simulink model "estimator"  (R2025b)
settings: configuration reference "cfgEstimator" (kept outside this file)
undefined symbols (not defined in the file or in its folder): BMS_iRest, BMS_ocvSoc, BMS_ocvV, BMS_Qnom, BMS_socMismatchTol, BMS_tRelax, BMS_tRestRecal, BMS_Ts
libraries: simulink x4
settings Model: DataDictionary=estimator.sldd  Creator=SC-Br  LastModifiedBy=SC-Br
settings ConfigSetRef: SourceName=cfgEstimator

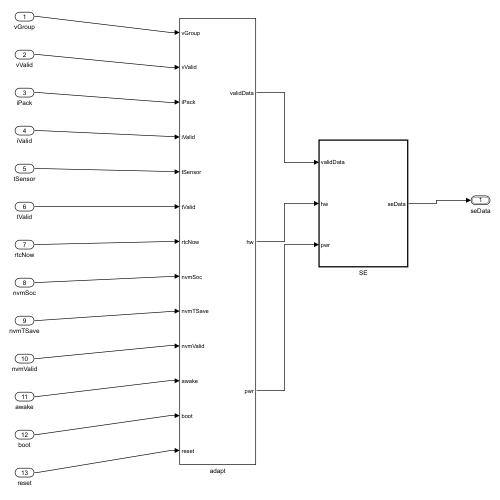
[thumbnail: Simulink's stored preview of the top-level diagram]
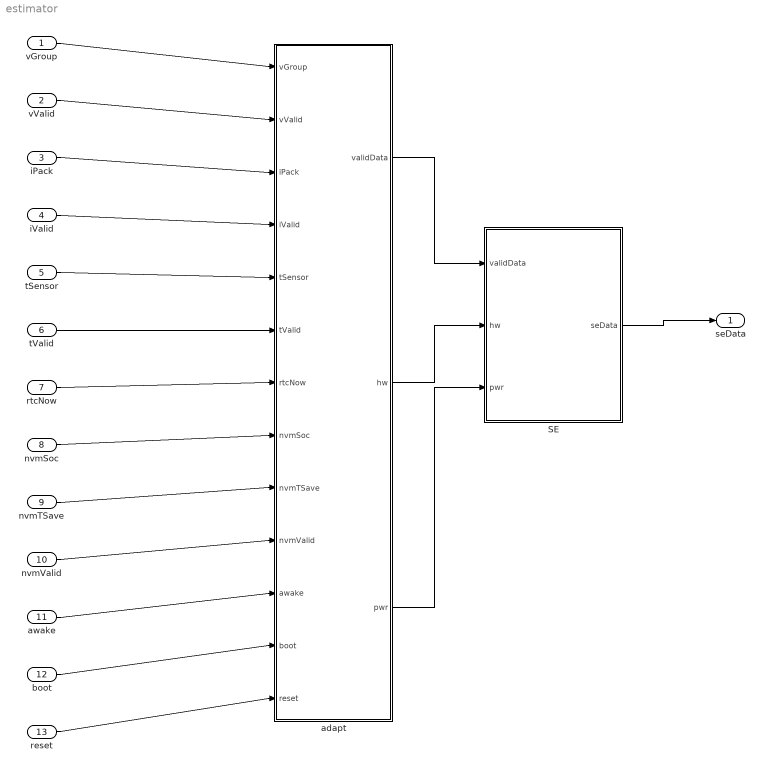
== system estimator ==
  vGroup : Inport  Description=Group voltages from f_CellVoltages (V)  OutDataTypeStr=double  PortDimensions=13  SampleTime=BMS_Ts
  vValid : Inport  Description=Not f_CellVoltages invalid flag  Port=2  OutDataTypeStr=boolean  PortDimensions=13  SampleTime=BMS_Ts
  iPack : Inport  Description=Pack current from f_PackValuesP0 (A, discharge positive)  Port=3  OutDataTypeStr=double  PortDimensions=1  SampleTime=BMS_Ts
  iValid : Inport  Description=Current received and plausible  Port=4  OutDataTypeStr=boolean  PortDimensions=1  SampleTime=BMS_Ts
  tSensor : Inport  Description=Temperatures from f_CellTemperatures (K)  Port=5  OutDataTypeStr=double  PortDimensions=26  SampleTime=BMS_Ts
  tValid : Inport  Description=Not f_CellTemperatures invalid flag  Port=6  OutDataTypeStr=boolean  PortDimensions=26  SampleTime=BMS_Ts
  rtcNow : Inport  Description=Pi clock (s, same epoch as nvmTSave)  Port=7  OutDataTypeStr=double  PortDimensions=1  SampleTime=BMS_Ts
  nvmSoc : Inport  Description=SOC record file: group SOC  Port=8  OutDataTypeStr=double  PortDimensions=13  SampleTime=BMS_Ts
  nvmTSave : Inport  Description=SOC record file: save time (s)  Port=9  OutDataTypeStr=double  PortDimensions=1  SampleTime=BMS_Ts
  nvmValid : Inport  Description=SOC record file present and intact  Port=10  OutDataTypeStr=boolean  PortDimensions=1  SampleTime=BMS_Ts
  awake : Inport  Description=BMS frames arriving (BMS on)  Port=11  OutDataTypeStr=boolean  PortDimensions=1  SampleTime=BMS_Ts
  boot : Inport  Description=One step: first measurement set after the BMS came on  Port=12  OutDataTypeStr=boolean  PortDimensions=1  SampleTime=BMS_Ts
  reset : Inport  Description=One step: SOC to be re-initialised from OCV  Port=13  OutDataTypeStr=boolean  PortDimensions=1  SampleTime=BMS_Ts
  SE : Subsystem  TreatAsAtomicUnit=on  RTWFcnName=SE_Step
      settings: RTWSystemCode=Nonreusable function  RTWFcnNameOpts=User specified  RTWFileNameOpts=Use function name
  adapt : Subsystem
  seData : Outport  OutDataTypeStr=Bus: BMS_seData
  wires:
  vGroup/1 -> adapt/1(vGroup)
  vValid/1 -> adapt/2(vValid)
  iPack/1 -> adapt/3(iPack)
  iValid/1 -> adapt/4(iValid)
  tSensor/1 -> adapt/5(tSensor)
  tValid/1 -> adapt/6(tValid)
  rtcNow/1 -> adapt/7(rtcNow)
  nvmSoc/1 -> adapt/8(nvmSoc)
  nvmTSave/1 -> adapt/9(nvmTSave)
  nvmValid/1 -> adapt/10(nvmValid)
  awake/1 -> adapt/11(awake)
  boot/1 -> adapt/12(boot)
  reset/1 -> adapt/13(reset)
  adapt/1(validData) -> SE/1(validData)
  adapt/2(hw) -> SE/2(hw)
  adapt/3(pwr) -> SE/3(pwr)
  SE/1(seData) -> seData/1

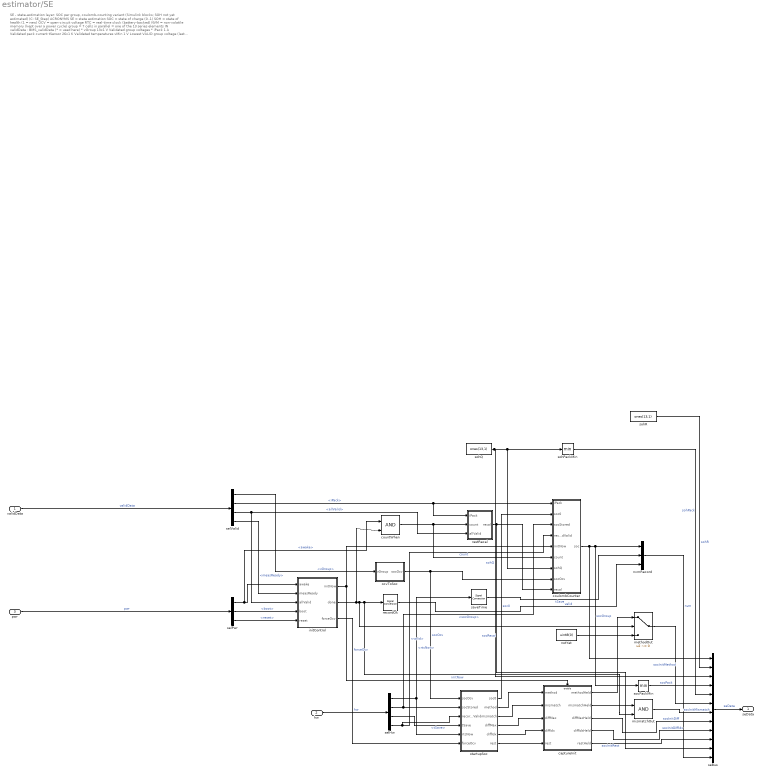
== system estimator/SE ==
  note: SE - state-estimation layer: SOC per group, coulomb-counting variant (Simulink blocks; SOH not yet estimated)   (C: SE_Step)
      |
      | ACRONYMS
      |   SE = state estimation
      |   SOC = state of charge (0..1)
      |   SOH = state of health (1 = new)
      |   OCV = open-circuit voltage
      |   RTC = real-time clock (battery-backed)
      |   NVM = non-volatile memory (kept over a power cycle)
      |   group = 7 cells in parallel = one of the 13 series elements
      |
      | IN   validData : BMS_validData   (* = used here)
      |   * vGroup         13x1  V     Validated group voltages
      |   * iPack          1     A     Validated pack current
      |     tSensor        26x1  K     Validated temperatures
      |     vMin           1     V     Lowest VALID group voltage (last valid value held if none valid)
      |     vMax           1     V     Highest VALID group voltage (last valid value held if none valid)
      |     tMin           1     K     Lowest VALID temperature (last valid value held if none valid)
      |     tMax           1     K     Highest VALID temperature (last valid value held if none valid)
      |   * allValid       1     bool  Every channel plausible
      |     contactorFb    1     bool  Validated main contactor feedback: true = closed
      |   * measReady      1     bool  Every sensor type has delivered a new sample since start-up (latched)
      |     vMinIdx        1     -     Group (1-13) with the lowest valid voltage; 0 = none valid yet
      |     vMaxIdx        1     -     Group (1-13) with the highest valid voltage; 0 = none valid yet
      |     tMinIdx        1     -     Sensor (1-26) with the lowest valid temperature; 0 = none valid yet
      |     tMaxIdx        1     -     Sensor (1-26) with the highest valid temperature; 0 = none valid yet
      |
      | IN   hw : BMS_hwIn   (* = used here)
      |   * rtcNow         1     s     Real-time clock now (battery-backed; keeps time while the BMS is off)
      |   * nvm            1     -     Record read from non-volatile memory at power-up
      |     powerBtn       1     bool  Power button pressed (long press BMS_tPowerPress: on / off)
      |     resetBtn       1     bool  Reset button pressed (long press BMS_tResetPress: restart, SOC from OCV)
      |
      | IN   pwr : BMS_pwrData   (* = used here)
      |   * awake          1     bool  BMS on (woken by a power long press, until the next one)
      |   * boot           1     bool  One-step pulse: every layer restarts as after a power-up (wake or reset)
      |   * reset          1     bool  One-step pulse: reset long press (SOC from OCV, ERROR latch cleared)
      |     powerOn        1     bool  One-step pulse: woken by the power button
      |     powerOff       1     bool  One-step pulse: switched off by the power button
      |
      | PARAMETERS (bms.sldd)
      |   BMS_ocvSoc       = [0 0.1 0.2 0.3 0.4 0.5 0.6 0.7 0.8 0.9 1] 1   SOC breakpoints of the BMS OCV table (placeholder)
      |   BMS_ocvV         = [2.65 3.38 3.51 3.59 3.655 3.725 3.795 3.875 3.97 4.075 4.2] V   Cell (= group) OCV at BMS_ocvSoc, strictly increasing (placeholder)
      |   BMS_Qnom         = 23.45 A*h   Nominal (new) parallel-group capacity Q_nom: 7 cells x 3.35 Ah (placeholder). Actual capacity per group Q_act = BMS_Qnom * SOH_Q, used by coulomb counting.
      |   BMS_tRelax       = 7200 s   Rest time since switch-off after which OCV is used at start-up (cells relaxed); shorter rests keep the stored SOC (placeholder)
      |   BMS_socMismatchTol = 0.1 1   Largest stored-vs-OCV SOC difference explained by OCV error; beyond it the battery is taken as recharged or swapped while off and OCV is used
      |   BMS_iRest        = 0.2 A   Current magnitude below which the pack is at rest: no charge temperature window (SOA), rest timer for SOC recalibration (SE) (foxBMS default 200 mA)
      |   BMS_tRestRecal   = 600 s   Time at rest (|iPack| < BMS_iRest, switch closed, all valid) after which SOC is set from OCV while the rest lasts (foxBMS example: 10 min; placeholder)
      |   BMS_Ts           = 0.1 s   BMS task period: the rate at which the BMS reads its inputs and runs MEAS..BMS (must be a multiple of the 10 ms base rate in cfgBMS)
      |
      | OUT  seData : BMS_seData
      |     socGroup       13x1  1     Estimated group SOC, 0-1
      |     sohR           13x1  1     Resistance SOH per group (1 = new)
      |     sohQ           13x1  1     Capacity SOH per group (1 = new)
      |     socPack        1     1     Pack SOC (minimum group SOC)
      |     sohPack        1     1     Pack SOH (worst group)
      |     socInitMethod  1     -     How SOC was initialised: 0 not yet, 1 stored, 3 OCV (2 not used)
      |     socInitMismatch 1     bool  Stored SOC disagreed with OCV beyond BMS_socMismatchTol (OCV used)
      |     socInitDiff    1     1     Largest |stored - OCV| SOC difference over the groups at initialisation
      |     socInitDiffIdx 1     -     Group (1-13) with that largest difference; 0 = not evaluated
      |     socInitRest    1     s     Rest time since the stored record was saved (rtcNow - tSave); -1 = no stored record used (none valid, or reset)
      |     socRecal       1     bool  SOC being recalibrated from OCV: pack at rest (|iPack| < BMS_iRest) for BMS_tRestRecal
      |     nvm            1     -     Record to save (current SOC, time, valid once SOC is initialised)
      |
      | WHAT IT DOES
      |   - Blocks: ocvToSoc -> startupSoc (decision) | initControl (when) | restRecal (rest timer) | coulombCounter | captureInit (holds result)
      |   - Start-up, after every power-on or reset, on the first step with every measurement valid (switch open):
      |     socOcv = OCV-table inverse of each group voltage; rest = rtcNow - nvm.tSave
      |     record invalid or rest < 0 -> OCV | |stored - OCV| > BMS_socMismatchTol on any group
      |     (recharged or swapped while off) -> OCV, flagged | reset or rest >= BMS_tRelax -> OCV | else stored SOC
      |   - Then coulomb counting: SOC -= iPack * Ts / (3600 * BMS_Qnom * sohQ), limited to 0..1
      |   - At rest (as foxBMS): |iPack| < BMS_iRest for BMS_tRestRecal -> SOC = OCV while the rest lasts (socRecal)
      |   - socPack = lowest group SOC; nvm = record to save (valid once SOC is initialised)
      |
      | LIMITATIONS / LATER
      |   - sohR and sohQ are constant 1: NO state-of-health estimation yet (placeholders); OCV table and BMS_tRelax are placeholders
      |   - A stored-SOC error smaller than BMS_socMismatchTol is kept after a short rest; EKF / RLS variants later
      |   - At-rest OCV is the terminal voltage under the hotel load (< BMS_iRest): small IR error, as foxBMS
  validData : Inport  OutDataTypeStr=Bus: BMS_validData
  hw : Inport  Port=2  OutDataTypeStr=Bus: BMS_hwIn
  pwr : Inport  Port=3  OutDataTypeStr=Bus: BMS_pwrData
  captureInit : Subsystem
  coulombCounter : Subsystem
  countWhen : Logic  IconShape=distinctive
  initControl : Subsystem
  methodOut : Switch  Criteria=u2 ~= 0
  mismatchOut : Logic  IconShape=distinctive
  notYet : Constant  Value=uint8(0)
  nvmRecord : BusCreator  Inputs=3  OutDataTypeStr=Bus: BMS_nvmRecord
  ocvToSoc : Subsystem
  recordOk : SignalConversion  OverrideOpt=off
  restRecal : Subsystem
  saveTime : SignalConversion  OverrideOpt=off
  seBus : BusCreator  Inputs=12  OutDataTypeStr=Bus: BMS_seData
  selHw : BusSelector  OutputSignals=rtcNow,nvm.socGroup,nvm.tSave,nvm.valid
  selPwr : BusSelector  OutputSignals=awake,boot,reset
  selValid : BusSelector  OutputSignals=vGroup,iPack,allValid,measReady
  socPackMin : MinMax
  sohPackMin : MinMax
  sohQ : Constant  Value=ones(13,1)
  sohR : Constant  Value=ones(13,1)
  startupSoc : Subsystem
  seData : Outport  OutDataTypeStr=Bus: BMS_seData
  wires:
  seBus/1 -> seData/1  "seData"
  captureInit/5(restHeld) -> seBus/10  "socInitRest"
  captureInit/4(diffIdxHeld) -> seBus/9  "socInitDiffIdx"
  captureInit/3(diffMaxHeld) -> seBus/8  "socInitDiff"
  mismatchOut/1 -> seBus/7  "socInitMismatch"
  methodOut/1 -> seBus/6  "socInitMethod"
  sohPackMin/1 -> seBus/5  "sohPack"
  socPackMin/1 -> seBus/4  "socPack"
  sohR/1 -> seBus/2  "sohR"
  recordOk/1 -> nvmRecord/3  "valid"
  saveTime/1 -> nvmRecord/2  "tSave"
  coulombCounter/1(soc) -> seBus/1, nvmRecord/1, socPackMin/1  "socGroup"
  captureInit/2(mismatchHeld) -> mismatchOut/1
  notYet/1 -> methodOut/3
  captureInit/1(methodHeld) -> methodOut/1
  startupSoc/6(rest) -> captureInit/5(rest)
  startupSoc/5(diffIdx) -> captureInit/4(diffIdx)
  startupSoc/4(diffMax) -> captureInit/3(diffMax)
  startupSoc/3(mismatch) -> captureInit/2(mismatch)
  startupSoc/2(method) -> captureInit/1(method)
  sohQ/1 -> seBus/3, sohPackMin/1, coulombCounter/7(sohQ)  "sohQ"
  countWhen/1 -> coulombCounter/6(count), restRecal/2(count)  "count"
  initControl/1(initNow) -> captureInit/Enable, coulombCounter/5(initNow)  "initNow"
  startupSoc/1(soc0) -> coulombCounter/2(soc0)  "soc0"
  selValid/2 -> coulombCounter/1(iPack), restRecal/1(iPack)  "<iPack>"
  initControl/2(done) -> countWhen/2, methodOut/2, recordOk/1, mismatchOut/2
  initControl/3(forceOcv) -> startupSoc/6(forceOcv)  "forceOcv"
  selHw/1 -> saveTime/1, startupSoc/5(rtcNow)  "<rtcNow>"
  selHw/3 -> startupSoc/4(tSave)  "<tSave>"
  selHw/4 -> coulombCounter/4(recordValid), startupSoc/3(recordValid)  "<valid>"
  selHw/2 -> coulombCounter/3(socStored), startupSoc/2(socStored)  "<socGroup>"
  ocvToSoc/1(socOcv) -> startupSoc/1(socOcv), coulombCounter/8(socOcv)  "socOcv"
  selPwr/3 -> initControl/5(reset)  "<reset>"
  selPwr/2 -> initControl/4(boot)  "<boot>"
  selValid/3 -> initControl/3(allValid), restRecal/3(allValid)  "<allValid>"
  selValid/4 -> initControl/2(measReady)  "<measReady>"
  selPwr/1 -> countWhen/1, initControl/1(awake)  "<awake>"
  selValid/1 -> ocvToSoc/1(vGroup)  "<vGroup>"
  pwr/1 -> selPwr/1  "pwr"
  hw/1 -> selHw/1  "hw"
  validData/1 -> selValid/1  "validData"
  restRecal/1(recal) -> coulombCounter/9(recal), seBus/11  "socRecal"
  nvmRecord/1 -> seBus/12  "nvm"

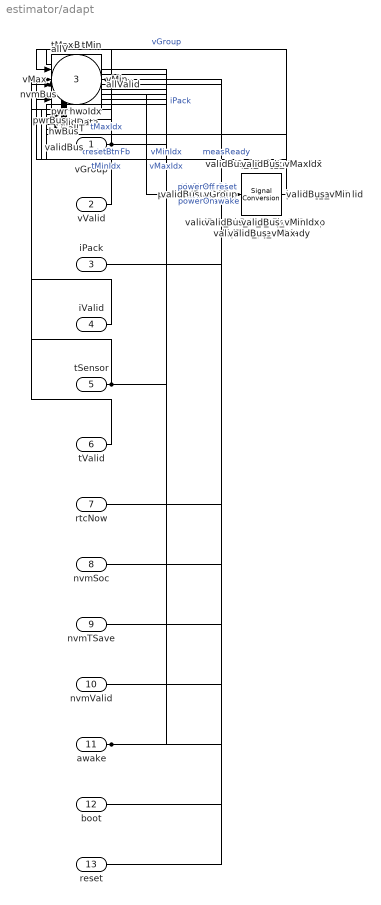
== system estimator/adapt ==
  vGroup : Inport
  vValid : Inport  Port=2
  iPack : Inport  Port=3
  iValid : Inport  Port=4
  tSensor : Inport  Port=5
  tValid : Inport  Port=6
  rtcNow : Inport  Port=7
  nvmSoc : Inport  Port=8
  nvmTSave : Inport  Port=9
  nvmValid : Inport  Port=10
  awake : Inport  Port=11
  boot : Inport  Port=12
  reset : Inport  Port=13
  allT : Logic  Inputs=1
  allV : Logic  Inputs=1
  allValid : Logic  Inputs=3
  hwBus : BusCreator  Inputs=4  OutDataTypeStr=Bus: BMS_hwIn
  hwBus_nvm : SignalConversion  OverrideOpt=off
  hwBus_powerBtn : SignalConversion  OverrideOpt=off
  hwBus_resetBtn : SignalConversion  OverrideOpt=off
  hwBus_rtcNow : SignalConversion  OverrideOpt=off
  noBtn : Constant  Value=false  OutDataTypeStr=boolean
  noFb : Constant  Value=false  OutDataTypeStr=boolean
  noIdx : Constant  Value=uint8(0)  OutDataTypeStr=uint8
  nvmBus : BusCreator  Inputs=3  OutDataTypeStr=Bus: BMS_nvmRecord
  nvmBus_socGroup : SignalConversion  OverrideOpt=off
  nvmBus_tSave : SignalConversion  OverrideOpt=off
  nvmBus_valid : SignalConversion  OverrideOpt=off
  pwrBus : BusCreator  Inputs=5  OutDataTypeStr=Bus: BMS_pwrData
  pwrBus_awake : SignalConversion  OverrideOpt=off
  pwrBus_boot : SignalConversion  OverrideOpt=off
  pwrBus_powerOff : SignalConversion  OverrideOpt=off
  pwrBus_powerOn : SignalConversion  OverrideOpt=off
  pwrBus_reset : SignalConversion  OverrideOpt=off
  tMax : MinMax  Function=max
  tMin : MinMax
  vMax : MinMax  Function=max
  vMin : MinMax
  validBus : BusCreator  Inputs=14  OutDataTypeStr=Bus: BMS_validData
  validBus_allValid : SignalConversion  OverrideOpt=off
  validBus_contactorFb : SignalConversion  OverrideOpt=off
  validBus_iPack : SignalConversion  OverrideOpt=off
  validBus_measReady : SignalConversion  OverrideOpt=off
  validBus_tMax : SignalConversion  OverrideOpt=off
  validBus_tMaxIdx : SignalConversion  OverrideOpt=off
  validBus_tMin : SignalConversion  OverrideOpt=off
  validBus_tMinIdx : SignalConversion  OverrideOpt=off
  validBus_tSensor : SignalConversion  OverrideOpt=off
  validBus_vGroup : SignalConversion  OverrideOpt=off
  validBus_vMax : SignalConversion  OverrideOpt=off
  validBus_vMaxIdx : SignalConversion  OverrideOpt=off
  validBus_vMin : SignalConversion  OverrideOpt=off
  validBus_vMinIdx : SignalConversion  OverrideOpt=off
  validData : Outport
  hw : Outport  Port=2
  pwr : Outport  Port=3
  wires:
  vGroup/1 -> vMin/1, vMax/1, validBus_vGroup/1
  tSensor/1 -> tMin/1, tMax/1, validBus_tSensor/1
  vValid/1 -> allV/1
  tValid/1 -> allT/1
  allV/1 -> allValid/1
  iValid/1 -> allValid/2
  allT/1 -> allValid/3
  validBus_vGroup/1 -> validBus/1  "vGroup"
  iPack/1 -> validBus_iPack/1
  validBus_iPack/1 -> validBus/2  "iPack"
  validBus_tSensor/1 -> validBus/3  "tSensor"
  vMin/1 -> validBus_vMin/1
  validBus_vMin/1 -> validBus/4  "vMin"
  vMax/1 -> validBus_vMax/1
  validBus_vMax/1 -> validBus/5  "vMax"
  tMin/1 -> validBus_tMin/1
  validBus_tMin/1 -> validBus/6  "tMin"
  tMax/1 -> validBus_tMax/1
  validBus_tMax/1 -> validBus/7  "tMax"
  allValid/1 -> validBus_allValid/1
  validBus_allValid/1 -> validBus/8  "allValid"
  noFb/1 -> validBus_contactorFb/1
  validBus_contactorFb/1 -> validBus/9  "contactorFb"
  awake/1 -> validBus_measReady/1, pwrBus_awake/1
  validBus_measReady/1 -> validBus/10  "measReady"
  noIdx/1 -> validBus_vMinIdx/1, validBus_vMaxIdx/1, validBus_tMinIdx/1, validBus_tMaxIdx/1
  validBus_vMinIdx/1 -> validBus/11  "vMinIdx"
  validBus_vMaxIdx/1 -> validBus/12  "vMaxIdx"
  validBus_tMinIdx/1 -> validBus/13  "tMinIdx"
  validBus_tMaxIdx/1 -> validBus/14  "tMaxIdx"
  validBus/1 -> validData/1
  nvmSoc/1 -> nvmBus_socGroup/1
  nvmBus_socGroup/1 -> nvmBus/1  "socGroup"
  nvmTSave/1 -> nvmBus_tSave/1
  nvmBus_tSave/1 -> nvmBus/2  "tSave"
  nvmValid/1 -> nvmBus_valid/1
  nvmBus_valid/1 -> nvmBus/3  "valid"
  rtcNow/1 -> hwBus_rtcNow/1
  hwBus_rtcNow/1 -> hwBus/1  "rtcNow"
  nvmBus/1 -> hwBus_nvm/1
  hwBus_nvm/1 -> hwBus/2  "nvm"
  noBtn/1 -> hwBus_powerBtn/1, hwBus_resetBtn/1, pwrBus_powerOn/1, pwrBus_powerOff/1
  hwBus_powerBtn/1 -> hwBus/3  "powerBtn"
  hwBus_resetBtn/1 -> hwBus/4  "resetBtn"
  hwBus/1 -> hw/1
  pwrBus_awake/1 -> pwrBus/1  "awake"
  boot/1 -> pwrBus_boot/1
  pwrBus_boot/1 -> pwrBus/2  "boot"
  reset/1 -> pwrBus_reset/1
  pwrBus_reset/1 -> pwrBus/3  "reset"
  pwrBus_powerOn/1 -> pwrBus/4  "powerOn"
  pwrBus_powerOff/1 -> pwrBus/5  "powerOff"
  pwrBus/1 -> pwr/1

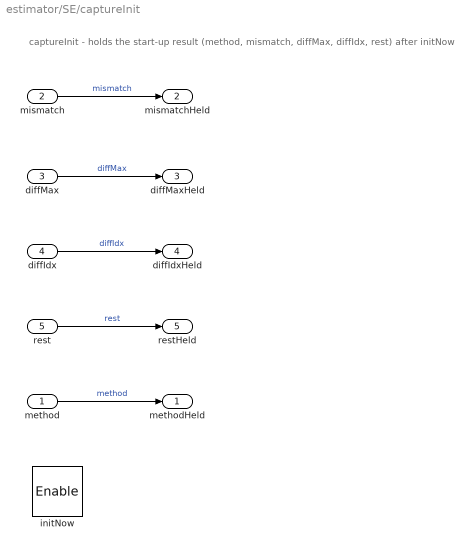
== system estimator/SE/captureInit ==
  note: captureInit - holds the start-up result (method, mismatch, diffMax, diffIdx, rest) after initNow
  method : Inport
  mismatch : Inport  Port=2
  diffMax : Inport  Port=3
  diffIdx : Inport  Port=4
  rest : Inport  Port=5
  initNow : EnablePort
  methodHeld : Outport  InitialOutput=0
  mismatchHeld : Outport  Port=2  InitialOutput=0
  diffMaxHeld : Outport  Port=3  InitialOutput=0
  diffIdxHeld : Outport  Port=4  InitialOutput=0
  restHeld : Outport  Port=5  InitialOutput=0
  wires:
  method/1 -> methodHeld/1  "method"
  mismatch/1 -> mismatchHeld/1  "mismatch"
  diffMax/1 -> diffMaxHeld/1  "diffMax"
  diffIdx/1 -> diffIdxHeld/1  "diffIdx"
  rest/1 -> restHeld/1  "rest"

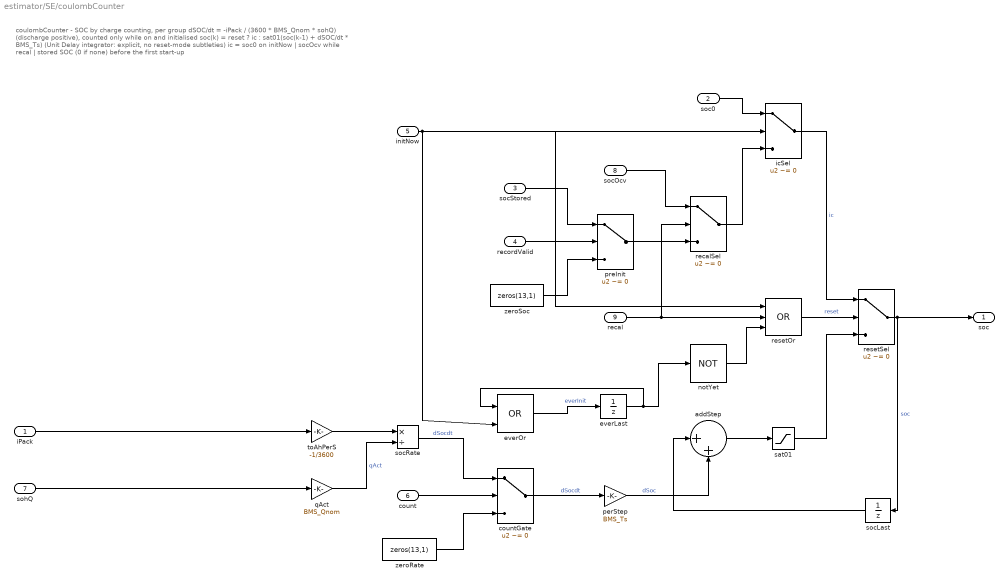
== system estimator/SE/coulombCounter ==
  note: coulombCounter - SOC by charge counting, per group
      |   dSOC/dt = -iPack / (3600 * BMS_Qnom * sohQ)  (discharge positive), counted only while on and initialised
      |   soc(k) = reset ? ic : sat01(soc(k-1) + dSOC/dt * BMS_Ts)   (Unit Delay integrator: explicit, no reset-mode subtleties)
      |   ic = soc0 on initNow | socOcv while recal | stored SOC (0 if none) before the first start-up
  iPack : Inport
  soc0 : Inport  Port=2
  socStored : Inport  Port=3
  recordValid : Inport  Port=4
  initNow : Inport  Port=5
  count : Inport  Port=6
  sohQ : Inport  Port=7
  socOcv : Inport  Port=8
  recal : Inport  Port=9
  addStep : Sum  Inputs=|++
  countGate : Switch  Criteria=u2 ~= 0
  everLast : UnitDelay  InitialCondition=false  SampleTime=-1
  everOr : Logic  Operator=OR  IconShape=distinctive
  icSel : Switch  Criteria=u2 ~= 0
  notYet : Logic  Operator=NOT  IconShape=distinctive
  perStep : Gain  Gain=BMS_Ts
  preInit : Switch  Criteria=u2 ~= 0
  qAct : Gain  Gain=BMS_Qnom
  recalSel : Switch  Criteria=u2 ~= 0
  resetOr : Logic  Operator=OR  Inputs=3  IconShape=distinctive
  resetSel : Switch  Criteria=u2 ~= 0
  sat01 : Saturate  UpperLimit=1  LowerLimit=0
  socLast : UnitDelay  SampleTime=-1
  socRate : Product  Inputs=*/
  toAhPerS : Gain  Gain=-1/3600
  zeroRate : Constant  Value=zeros(13,1)
  zeroSoc : Constant  Value=zeros(13,1)
  soc : Outport
  wires:
  recalSel/1 -> icSel/3
  preInit/1 -> recalSel/3
  recal/1 -> recalSel/2, resetOr/2
  socOcv/1 -> recalSel/1
  iPack/1 -> toAhPerS/1
  sohQ/1 -> qAct/1
  toAhPerS/1 -> socRate/1
  qAct/1 -> socRate/2  "qAct"
  socRate/1 -> countGate/1  "dSocdt"
  count/1 -> countGate/2
  zeroRate/1 -> countGate/3
  socStored/1 -> preInit/1
  recordValid/1 -> preInit/2
  zeroSoc/1 -> preInit/3
  soc0/1 -> icSel/1
  initNow/1 -> icSel/2, everOr/2, resetOr/1
  countGate/1 -> perStep/1  "dSocdt"
  socLast/1 -> addStep/1
  perStep/1 -> addStep/2  "dSoc"
  addStep/1 -> sat01/1
  icSel/1 -> resetSel/1  "ic"
  sat01/1 -> resetSel/3
  resetSel/1 -> soc/1, socLast/1  "soc"
  everLast/1 -> everOr/1, notYet/1
  everOr/1 -> everLast/1  "everInit"
  notYet/1 -> resetOr/3
  resetOr/1 -> resetSel/2  "reset"

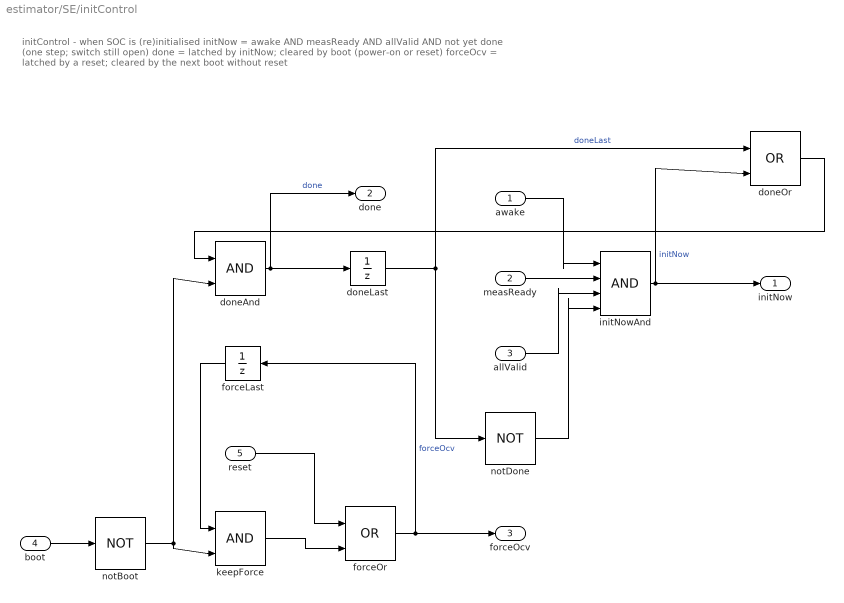
== system estimator/SE/initControl ==
  note: initControl - when SOC is (re)initialised
      |   initNow  = awake AND measReady AND allValid AND not yet done   (one step; switch still open)
      |   done     = latched by initNow; cleared by boot (power-on or reset)
      |   forceOcv = latched by a reset; cleared by the next boot without reset
  awake : Inport
  measReady : Inport  Port=2
  allValid : Inport  Port=3
  boot : Inport  Port=4
  reset : Inport  Port=5
  doneAnd : Logic  IconShape=distinctive
  doneLast : UnitDelay  InitialCondition=false  SampleTime=-1
  doneOr : Logic  Operator=OR  IconShape=distinctive
  forceLast : UnitDelay  InitialCondition=false  SampleTime=-1
  forceOr : Logic  Operator=OR  IconShape=distinctive
  initNowAnd : Logic  Inputs=4  IconShape=distinctive
  keepForce : Logic  IconShape=distinctive
  notBoot : Logic  Operator=NOT  IconShape=distinctive
  notDone : Logic  Operator=NOT  IconShape=distinctive
  initNow : Outport
  done : Outport  Port=2
  forceOcv : Outport  Port=3
  wires:
  doneLast/1 -> notDone/1, doneOr/1  "doneLast"
  awake/1 -> initNowAnd/1
  measReady/1 -> initNowAnd/2
  allValid/1 -> initNowAnd/3
  notDone/1 -> initNowAnd/4
  initNowAnd/1 -> initNow/1, doneOr/2  "initNow"
  boot/1 -> notBoot/1
  doneOr/1 -> doneAnd/1
  notBoot/1 -> doneAnd/2, keepForce/2
  doneAnd/1 -> done/1, doneLast/1  "done"
  forceLast/1 -> keepForce/1
  reset/1 -> forceOr/1
  keepForce/1 -> forceOr/2
  forceOr/1 -> forceOcv/1, forceLast/1  "forceOcv"

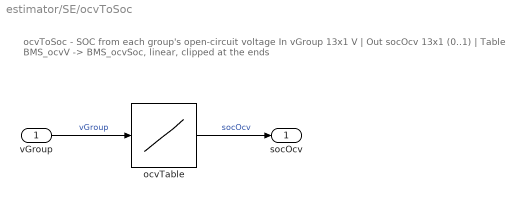
== system estimator/SE/ocvToSoc ==
  note: ocvToSoc - SOC from each group's open-circuit voltage
      |   In vGroup 13x1 V | Out socOcv 13x1 (0..1) | Table BMS_ocvV -> BMS_ocvSoc, linear, clipped at the ends
  vGroup : Inport
  ocvTable : Lookup_n-D  NumberOfTableDimensions=1  BreakpointsForDimension1=BMS_ocvV  Table=BMS_ocvSoc  ExtrapMethod=Clip  InternalRulePriority=Speed  RndMeth=Simplest
  socOcv : Outport
  wires:
  vGroup/1 -> ocvTable/1  "vGroup"
  ocvTable/1 -> socOcv/1  "socOcv"

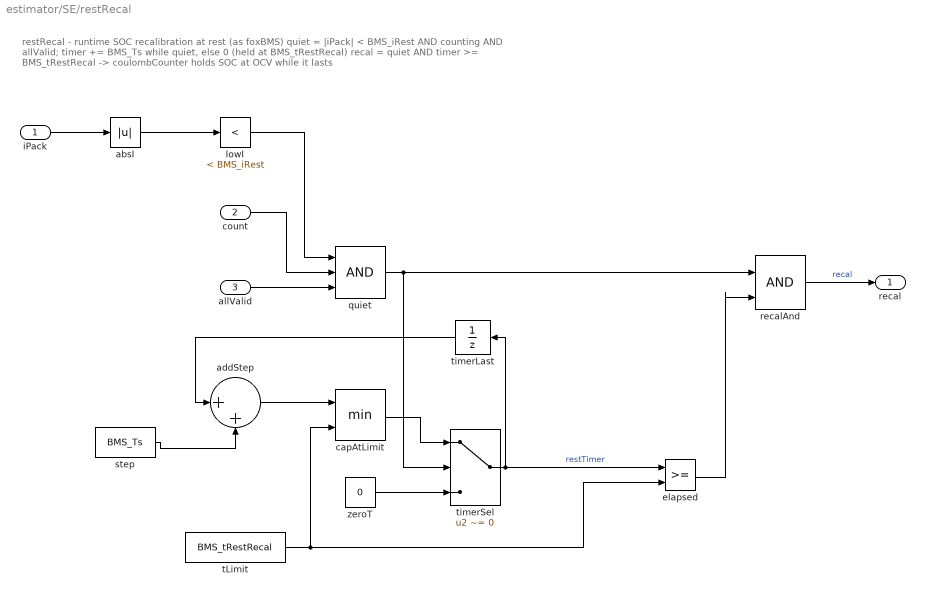
== system estimator/SE/restRecal ==
  note: restRecal - runtime SOC recalibration at rest (as foxBMS)
      |   quiet = |iPack| < BMS_iRest AND counting AND allValid;  timer += BMS_Ts while quiet, else 0 (held at BMS_tRestRecal)
      |   recal = quiet AND timer >= BMS_tRestRecal  ->  coulombCounter holds SOC at OCV while it lasts
  iPack : Inport
  count : Inport  Port=2
  allValid : Inport  Port=3
  absI : Abs
  addStep : Sum  Inputs=|++
  capAtLimit : MinMax  Inputs=2
  elapsed : RelationalOperator
  lowI : simulink/Logic and Bit Operations/Compare To Constant  relop=<  const=BMS_iRest  OutDataTypeStr=boolean
  quiet : Logic  Inputs=3  IconShape=distinctive
  recalAnd : Logic  IconShape=distinctive
  step : Constant  Value=BMS_Ts
  tLimit : Constant  Value=BMS_tRestRecal
  timerLast : UnitDelay  SampleTime=-1
  timerSel : Switch  Criteria=u2 ~= 0
  zeroT : Constant  Value=0
  recal : Outport
  wires:
  iPack/1 -> absI/1
  absI/1 -> lowI/1
  lowI/1 -> quiet/1
  count/1 -> quiet/2
  allValid/1 -> quiet/3
  timerLast/1 -> addStep/1
  step/1 -> addStep/2
  addStep/1 -> capAtLimit/1
  tLimit/1 -> capAtLimit/2, elapsed/2
  capAtLimit/1 -> timerSel/1
  quiet/1 -> timerSel/2, recalAnd/1
  zeroT/1 -> timerSel/3
  timerSel/1 -> timerLast/1, elapsed/1  "restTimer"
  elapsed/1 -> recalAnd/2
  recalAnd/1 -> recal/1  "recal"

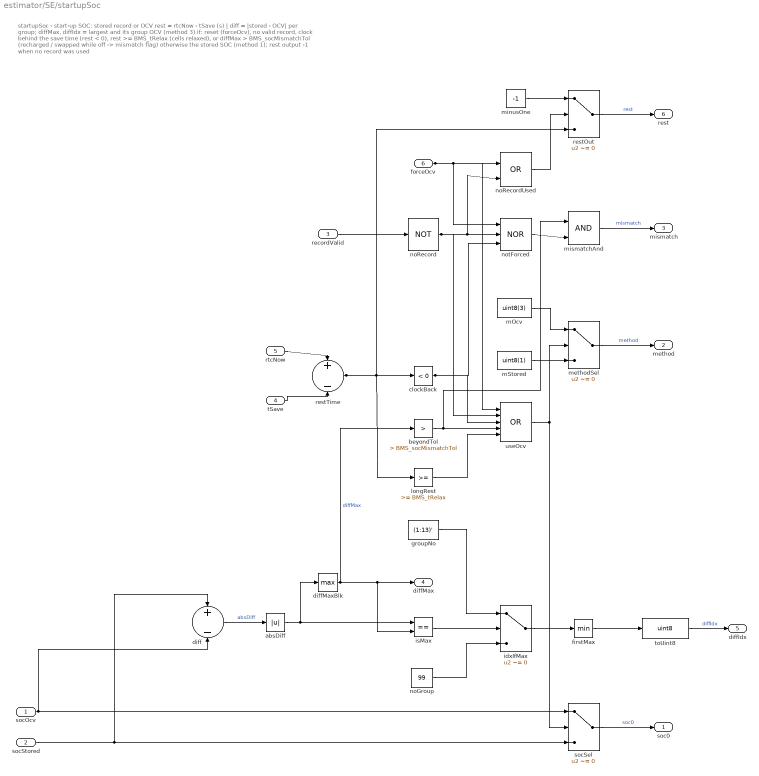
== system estimator/SE/startupSoc ==
  note: startupSoc - start-up SOC: stored record or OCV
      |   rest = rtcNow - tSave (s) | diff = |stored - OCV| per group; diffMax, diffIdx = largest and its group
      |   OCV (method 3) if: reset (forceOcv), no valid record, clock behind the save time (rest < 0),
      |      rest >= BMS_tRelax (cells relaxed), or diffMax > BMS_socMismatchTol (recharged / swapped while off -> mismatch flag)
      |   otherwise the stored SOC (method 1);  rest output -1 when no record was used
  socOcv : Inport
  socStored : Inport  Port=2
  recordValid : Inport  Port=3
  tSave : Inport  Port=4
  rtcNow : Inport  Port=5
  forceOcv : Inport  Port=6
  absDiff : Abs
  beyondTol : simulink/Logic and Bit Operations/Compare To Constant  relop=>  const=BMS_socMismatchTol  OutDataTypeStr=boolean
  clockBack : simulink/Logic and Bit Operations/Compare To Constant  relop=<  const=0  OutDataTypeStr=boolean
  diff : Sum  Inputs=+-
  diffMaxBlk : MinMax  Function=max
  firstMax : MinMax
  groupNo : Constant  Value=(1:13)'
  idxIfMax : Switch  Criteria=u2 ~= 0
  isMax : RelationalOperator  Operator===
  longRest : simulink/Logic and Bit Operations/Compare To Constant  relop=>=  const=BMS_tRelax  OutDataTypeStr=boolean
  mOcv : Constant  Value=uint8(3)
  mStored : Constant  Value=uint8(1)
  methodSel : Switch  Criteria=u2 ~= 0
  minusOne : Constant  Value=-1
  mismatchAnd : Logic  IconShape=distinctive
  noGroup : Constant  Value=99
  noRecord : Logic  Operator=NOT  IconShape=distinctive
  noRecordUsed : Logic  Operator=OR  IconShape=distinctive
  notForced : Logic  Operator=NOR  Inputs=3  IconShape=distinctive
  restOut : Switch  Criteria=u2 ~= 0
  restTime : Sum  Inputs=+-
  socSel : Switch  Criteria=u2 ~= 0
  toUint8 : DataTypeConversion  OutDataTypeStr=uint8
  useOcv : Logic  Operator=OR  Inputs=5  IconShape=distinctive
  soc0 : Outport
  method : Outport  Port=2
  mismatch : Outport  Port=3
  diffMax : Outport  Port=4
  diffIdx : Outport  Port=5
  rest : Outport  Port=6
  wires:
  restOut/1 -> rest/1  "rest"
  noRecordUsed/1 -> restOut/2
  minusOne/1 -> restOut/1
  mismatchAnd/1 -> mismatch/1  "mismatch"
  notForced/1 -> mismatchAnd/2
  beyondTol/1 -> mismatchAnd/1, useOcv/4
  clockBack/1 -> useOcv/3, notForced/3
  noRecord/1 -> noRecordUsed/2, notForced/2, useOcv/2
  forceOcv/1 -> notForced/1, useOcv/1, noRecordUsed/1
  recordValid/1 -> noRecord/1
  restTime/1 -> restOut/3, longRest/1, clockBack/1
  toUint8/1 -> diffIdx/1  "diffIdx"
  firstMax/1 -> toUint8/1
  idxIfMax/1 -> firstMax/1
  noGroup/1 -> idxIfMax/3
  isMax/1 -> idxIfMax/2
  groupNo/1 -> idxIfMax/1
  diffMaxBlk/1 -> isMax/2, diffMax/1, beyondTol/1  "diffMax"
  absDiff/1 -> diffMaxBlk/1, isMax/1
  diff/1 -> absDiff/1  "absDiff"
  socOcv/1 -> diff/2, socSel/1
  socStored/1 -> diff/1, socSel/3
  tSave/1 -> restTime/2
  rtcNow/1 -> restTime/1
  longRest/1 -> useOcv/5
  useOcv/1 -> socSel/2, methodSel/2
  socSel/1 -> soc0/1  "soc0"
  mOcv/1 -> methodSel/1
  mStored/1 -> methodSel/3
  methodSel/1 -> method/1  "method"
